simulink model "SR_ControlDiagram"  (R2024b)
settings: Solver=VariableStepAuto  StartTime=0.0  StopTime=10.0  RelTol=1e-3
undefined symbols (not defined in the file): d, i_lim, Ke, L, nd, R_fs, Rc, tau, Umax, v
settings Model: Creator=sange  LastModifiedBy=sange

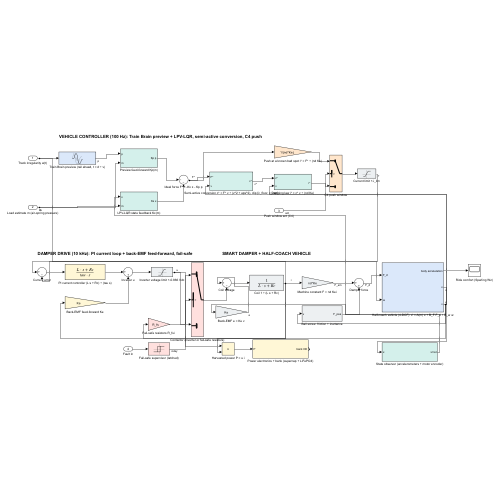
[thumbnail: Simulink's stored preview of the top-level diagram]
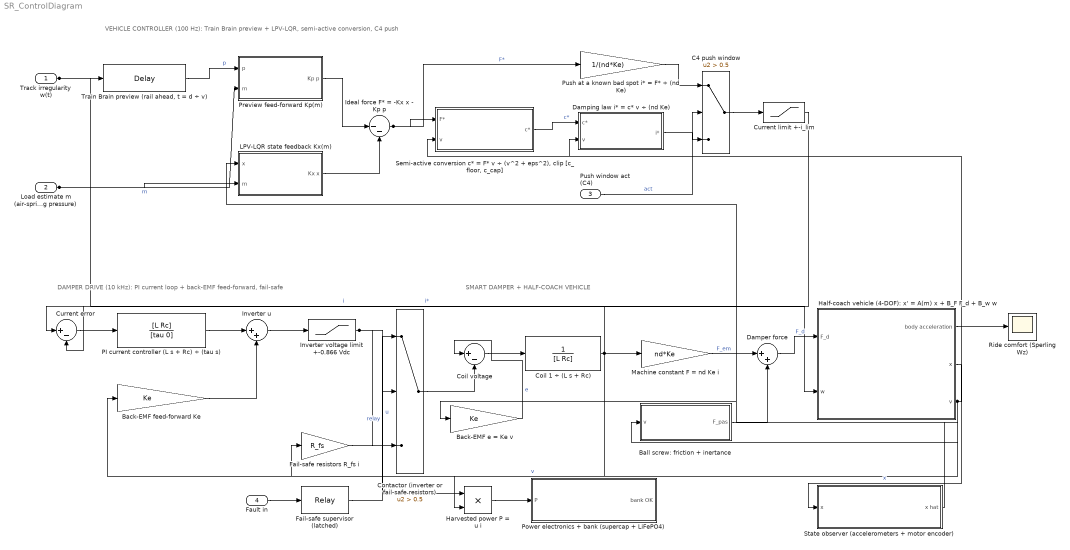
== system SR_ControlDiagram ==
  note: VEHICLE CONTROLLER (100 Hz): Train Brain preview + LPV-LQR, semi-active conversion, C4 push
  note: DAMPER DRIVE (10 kHz): PI current loop + back-EMF feed-forward, fail-safe
  note: SMART DAMPER + HALF-COACH VEHICLE
  Track irregularity w(t) : Inport
  Load estimate m (air-spring pressure) : Inport  Port=2
  Push window act (C4) : Inport  Port=3
  Fault in : Inport  Port=4
  Back-EMF e = Ke v : Gain  Gain=Ke
  Back-EMF feed-forward Ke : Gain  Gain=Ke
  Ball screw: friction + inertance : Subsystem
  C4 push window : Switch  Criteria=u2 > Threshold  Threshold=0.5  SaturateOnIntegerOverflow=off  InputSameDT=off
  Coil 1 ÷ (L s + Rc) : TransferFcn  Numerator=1  Denominator=[L Rc]
  Coil voltage : Sum  Inputs=|+-
  Contactor (inverter or fail-safe resistors) : Switch  Criteria=u2 > Threshold  Threshold=0.5  SaturateOnIntegerOverflow=off  InputSameDT=off
  Current error : Sum  Inputs=|+-
  Current limit +-i_lim : Saturate  UpperLimit=i_lim  LowerLimit=-i_lim
  Damper force : Sum  Inputs=|++
  Damping law i* = c* v ÷ (nd Ke) : Subsystem
  Fail-safe resistors R_fs i : Gain  Gain=R_fs
  Fail-safe supervisor (latched) : Relay  OnSwitchValue=0.5  OffSwitchValue=0.5
  Half-coach vehicle (4-DOF): x' = A(m) x + B_F F_d + B_w w : Subsystem
  Harvested power P = u i : Product
  Ideal force F* = -Kx x - Kp p : Sum  Inputs=|--
  Inverter u : Sum  Inputs=|++
  Inverter voltage limit +-0.866 Vdc : Saturate  UpperLimit=Umax  LowerLimit=-Umax
  LPV-LQR state feedback Kx(m) : Subsystem
  Machine constant F = nd Ke i : Gain  Gain=nd*Ke
  PI current controller (L s + Rc) ÷ (tau s) : TransferFcn  Numerator=[L Rc]  Denominator=[tau 0]
  Power electronics + bank (supercap + LiFePO4) : Subsystem
  Preview feed-forward Kp(m) : Subsystem
  Push at a known bad spot i* = F* ÷ (nd Ke) : Gain  Gain=1/(nd*Ke)
  Ride comfort (Sperling Wz) : Scope
  "Semi-active conversion c* = F* v ÷ (v^2 + eps^2), clip [c_floor, c_cap]" : Subsystem
  State observer (accelerometers + motor encoder) : Subsystem
  "Train Brain preview (rail ahead, t = d ÷ v)" : TransportDelay  DelayTime=d/v
  wires:
  Track irregularity w(t)/1 -> "Train Brain preview (rail ahead, t = d ÷ v)"/1, Half-coach vehicle (4-DOF): x' = A(m) x + B_F F_d + B_w w/2(w)
  "Train Brain preview (rail ahead, t = d ÷ v)"/1 -> Preview feed-forward Kp(m)/1(p)  "p"
  Load estimate m (air-spring pressure)/1 -> Preview feed-forward Kp(m)/2(m), LPV-LQR state feedback Kx(m)/2(m)  "m"
  Preview feed-forward Kp(m)/1(Kp p) -> Ideal force F* = -Kx x - Kp p/1
  LPV-LQR state feedback Kx(m)/1(Kx x) -> Ideal force F* = -Kx x - Kp p/2
  Ideal force F* = -Kx x - Kp p/1 -> "Semi-active conversion c* = F* v ÷ (v^2 + eps^2), clip [c_floor, c_cap]"/1(F*), Push at a known bad spot i* = F* ÷ (nd Ke)/1  "F*"
  "Semi-active conversion c* = F* v ÷ (v^2 + eps^2), clip [c_floor, c_cap]"/1(c*) -> Damping law i* = c* v ÷ (nd Ke)/1(c*)  "c*"
  Push at a known bad spot i* = F* ÷ (nd Ke)/1 -> C4 push window/1
  Push window act (C4)/1 -> C4 push window/2  "act"
  Damping law i* = c* v ÷ (nd Ke)/1(i*) -> C4 push window/3
  C4 push window/1 -> Current limit +-i_lim/1
  Current limit +-i_lim/1 -> Current error/1  "i*"
  Current error/1 -> PI current controller (L s + Rc) ÷ (tau s)/1
  PI current controller (L s + Rc) ÷ (tau s)/1 -> Inverter u/1
  Back-EMF feed-forward Ke/1 -> Inverter u/2
  Inverter u/1 -> Inverter voltage limit +-0.866 Vdc/1
  Inverter voltage limit +-0.866 Vdc/1 -> Contactor (inverter or fail-safe resistors)/3, Harvested power P = u i/1  "u"
  Fault in/1 -> Fail-safe supervisor (latched)/1
  Fail-safe supervisor (latched)/1 -> Contactor (inverter or fail-safe resistors)/2  "relay"
  Fail-safe resistors R_fs i/1 -> Contactor (inverter or fail-safe resistors)/1
  Contactor (inverter or fail-safe resistors)/1 -> Coil voltage/2
  Back-EMF e = Ke v/1 -> Coil voltage/1  "e"
  Coil voltage/1 -> Coil 1 ÷ (L s + Rc)/1
  Coil 1 ÷ (L s + Rc)/1 -> Machine constant F = nd Ke i/1, Current error/2, Fail-safe resistors R_fs i/1, Harvested power P = u i/2  "i"
  Harvested power P = u i/1 -> Power electronics + bank (supercap + LiFePO4)/1(P)
  Machine constant F = nd Ke i/1 -> Damper force/1  "F_em"
  Ball screw: friction + inertance/1(F_pas) -> Damper force/2
  Damper force/1 -> Half-coach vehicle (4-DOF): x' = A(m) x + B_F F_d + B_w w/1(F_d)  "F_d"
  Half-coach vehicle (4-DOF): x' = A(m) x + B_F F_d + B_w w/1(body acceleration) -> Ride comfort (Sperling Wz)/1
  Half-coach vehicle (4-DOF): x' = A(m) x + B_F F_d + B_w w/2(x) -> State observer (accelerometers + motor encoder)/1(x)  "x"
  State observer (accelerometers + motor encoder)/1(x hat) -> LPV-LQR state feedback Kx(m)/1(x)
  Half-coach vehicle (4-DOF): x' = A(m) x + B_F F_d + B_w w/3(v) -> "Semi-active conversion c* = F* v ÷ (v^2 + eps^2), clip [c_floor, c_cap]"/2(v), Damping law i* = c* v ÷ (nd Ke)/2(v), Back-EMF feed-forward Ke/1, Back-EMF e = Ke v/1, Ball screw: friction + inertance/1(v)  "v"

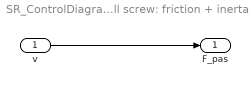
== system SR_ControlDiagram/Ball screw: friction + inertance ==
  v : Inport
  F_pas : Outport
  wires:
  v/1 -> F_pas/1

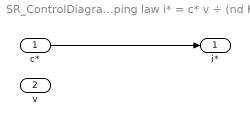
== system SR_ControlDiagram/Damping law i* = c* v ÷ (nd Ke) ==
  c* : Inport
  v : Inport  Port=2
  i* : Outport
  wires:
  c*/1 -> i*/1

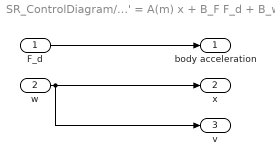
== system SR_ControlDiagram/Half-coach vehicle (4-DOF): x' = A(m) x + B_F F_d + B_w w ==
  F_d : Inport
  w : Inport  Port=2
  body acceleration : Outport
  x : Outport  Port=2
  v : Outport  Port=3
  wires:
  F_d/1 -> body acceleration/1
  w/1 -> x/1, v/1

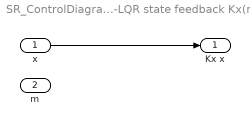
== system SR_ControlDiagram/LPV-LQR state feedback Kx(m) ==
  x : Inport
  m : Inport  Port=2
  Kx x : Outport
  wires:
  x/1 -> Kx x/1

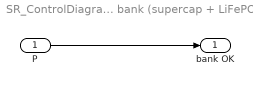
== system SR_ControlDiagram/Power electronics + bank (supercap + LiFePO4) ==
  P : Inport
  bank OK : Outport
  wires:
  P/1 -> bank OK/1

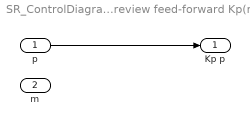
== system SR_ControlDiagram/Preview feed-forward Kp(m) ==
  p : Inport
  m : Inport  Port=2
  Kp p : Outport
  wires:
  p/1 -> Kp p/1

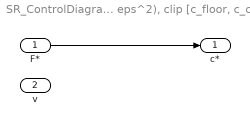
== system SR_ControlDiagram/Semi-active conversion c* = F* v ÷ (v^2 + eps^2), clip [c_floor, c_cap] ==
  F* : Inport
  v : Inport  Port=2
  c* : Outport
  wires:
  F*/1 -> c*/1

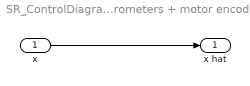
== system SR_ControlDiagram/State observer (accelerometers + motor encoder) ==
  x : Inport
  x hat : Outport
  wires:
  x/1 -> x hat/1
